simulink library "lib_Grid_AC_Static"  (R2026a)
settings: Solver=VariableStepAuto
undefined symbols (not defined in the file): iadmitt_matrix, Nbuses
settings Model: Creator=atomas  LastModifiedBy=atomas

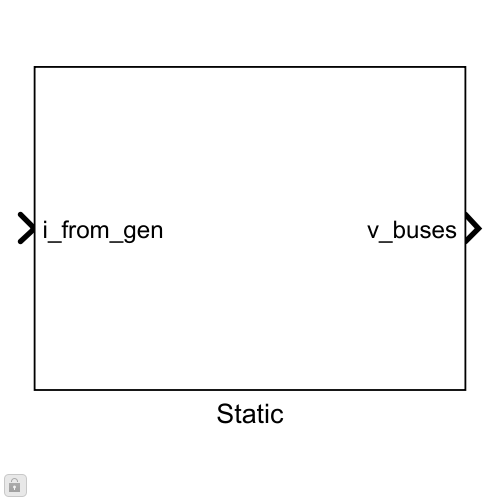
[thumbnail: Simulink's stored preview of the top-level diagram]
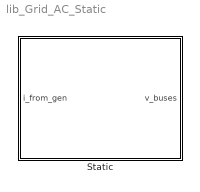
== system lib_Grid_AC_Static ==
  Static : Subsystem  VariantControl=Static

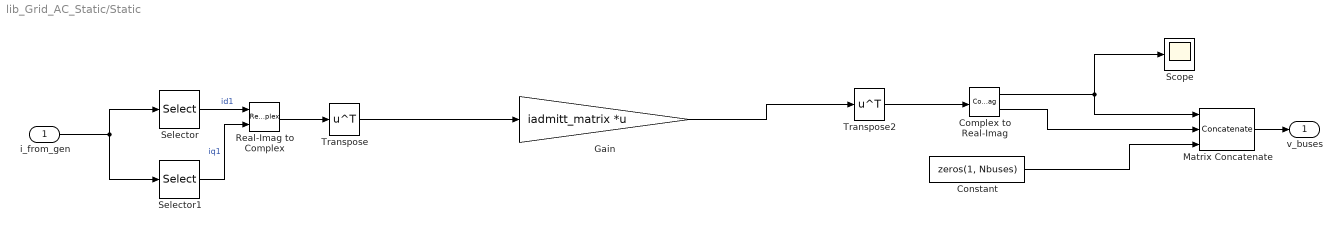
== system lib_Grid_AC_Static/Static ==
  i_from_gen : Inport
  Complex to Real-Imag : ComplexToRealImag
  Constant : Constant  Value=zeros(1, Nbuses)  VectorParams1D=off
  Gain : Gain  Gain=iadmitt_matrix  Multiplication=Matrix(K*u)
  Matrix Concatenate : Concatenate  NumInputs=3  Mode=Multidimensional array
  Real-Imag to Complex : RealImagToComplex
  Scope : Scope
      settings: ActiveDisplayYMinimum=1.0463  ActiveDisplayYMaximum=1.1306
  Selector : Selector  NumberOfDimensions=2  InputPortWidth=3  IndexOptions=Index vector (dialog),Select all  Indices=1,find(bus_complexity == 1)  OutputSizes=1,1
  Selector1 : Selector  NumberOfDimensions=2  InputPortWidth=3  IndexOptions=Index vector (dialog),Select all  Indices=2,find(bus_complexity == 1)  OutputSizes=1,1
  Transpose : Math  Operator=transpose
  Transpose2 : Math  Operator=transpose
  v_buses : Outport
  wires:
  Constant/1 -> Matrix Concatenate/3
  Selector/1 -> Real-Imag to Complex/1  "id1"
  Selector1/1 -> Real-Imag to Complex/2  "iq1"
  i_from_gen/1 -> Selector1/1, Selector/1
  Real-Imag to Complex/1 -> Transpose/1
  Complex to Real-Imag/1 -> Matrix Concatenate/1, Scope/1
  Complex to Real-Imag/2 -> Matrix Concatenate/2
  Transpose2/1 -> Complex to Real-Imag/1
  Transpose/1 -> Gain/1
  Gain/1 -> Transpose2/1
  Matrix Concatenate/1 -> v_buses/1
